simulink library "ConverterLibrary"  (R2026a)
settings: Solver=VariableStepAuto
undefined symbols (not defined in the file or in its folder): DiscIntNeverNeededParam, dspblkCoreblockFVToolHelper, gcbh, gridInverter
libraries: fl_lib x240, nesl_utility x221, ee_lib x208, slpidlib x28, eeGeneralControl x12, simulink x9, eeTransforms x4, simulink_extras x1, eePowerMeasurement x1
(part 3 of 30)

== system ConverterLibrary/Power Converter Plant/Power Factor Correction Converters ==
  Boost PFC Converter : Subsystem  mask(Boost PFC Converter){modelOption=Simplified, ratedPower=1000, ratedPower_unit=W, VIn=230, VIn_unit=V, FRated=50, FRated_unit=Hz, VOut=400, VOut_unit=V, Fsw=65000, Fsw_unit=Hz, LBoost=9.5731e-4, LBoost_unit=H, RLboost=0.05, RLboost_unit=Ohm, CBoost=7.9577e-4, CBoost_unit=F, Rco=0.01, Rco_unit=Ohm, Vco=380, Vco_unit=V, switchDeviceOption=MOSFET (Ideal, Switching) with Thermal, RdsOn=0.05, RdsOn_unit=Ohm, GdsOff=1e-5, GdsOff_unit=1/Ohm, Vth=3, Vth_unit=V, diodeDeviceOption=Tabulated Diode, VfDiode=0.6, VfDiode_unit=V, RdDiode=0.01, RdDiode_unit=Ohm, GdDiode=1e-5, GdDiode_unit=1/Ohm, rectDiodeDeviceOption=Tabulated Diode, VfRect=0.6, VfRect_unit=V, RdRect=0.3, RdRect_unit=Ohm, GdRect=1e-5, GdRect_unit=1/Ohm, VfPreCharge=0.6, VfPreCharge_unit=V, RdPreCharge=0.01, RdPreCharge_unit=Ohm, GdPreCharge=1e-5, GdPreCharge_unit=1/Ohm, RPreCharge=3, RPreCharge_unit=Ohm, simTemp=25, simTemp_unit=degC}
      mask prompts: modelOption "Boost PFC model option"; ratedPower "Rated power"; VIn "AC input voltage (RMS)"; FRated "Line frequency"; VOut "DC output voltage"; Fsw "Switching frequency"; LBoost "Boost inductance"; RLboost "Inductor resistance"; CBoost "Output capacitance"; Rco "Capacitor ESR"; Vco "Initial output capacitor voltage"; switchDeviceOption "Switch model"; RdsOn "On-state resistance"; GdsOff "Off-state conductance"; Vth "Threshold voltage"; diodeDeviceOption "Diode model"; VfDiode "Forward voltage"; RdDiode "On resistance"; GdDiode "Off conductance"; rectDiodeDeviceOption "Rectifier diode model"; VfRect "Forward voltage"; RdRect "On resistance"; GdRect "Off conductance"; VfPreCharge "Forward voltage"; RdPreCharge "On resistance"; GdPreCharge "Off conductance"; RPreCharge "Pre-charge resistance"; simTemp "Simulation temperature"
      mask help: Single-phase diode bridge + boost PFC power stage
      mask init:
      | %% Unit conversion: convert displayed values to base SI units
      | convMap = containers.Map( ...
      |     {'W','kW','MW','V','kV','mV','F','mF','uF','nF','pF', ...
      |      'H','mH','uH','nH','Ohm','kOhm','mOhm','S','mS','1/Ohm', ...
      |      'Hz','kHz','MHz'}, ...
      |     {1, 1e3, 1e6, 1, 1e3, 1e-3, 1, 1e-3, 1e-6, 1e-9, 1e-12, ...
      |      1, 1e-3, 1e-6, 1e-9, 1, 1e3, 1e-3, 1, 1e-3, 1, ...
      |      1, 1e3, 1e6});
      | 
      | ratedPower_SI = ratedPower * convMap(ratedPower_unit);
      | VIn_SI = VIn * convMap(VIn_unit);
      | FRated_SI = FRated * convMap(FRated_unit);
      | VOut_SI = VOut * convMap(VOut_unit);
      | Fsw_SI = Fsw * convMap(Fsw_unit);
      | LBoost_SI = LBoost * convMap(LBoost_unit);
      | RLboost_SI = RLboost * convMap(RLboost_unit);
      | CBoost_SI = CBoost * convMap(CBoost_unit);
      | Rco_SI = Rco * convMap(Rco_unit);
      | Vco_SI = Vco * convMap(Vco_unit);
      | RdsOn_SI = RdsOn * convMap(RdsOn_unit);
      | GdsOff_SI = GdsOff * convMap(GdsOff_unit);
      | Vth_SI = Vth * convMap(Vth_unit);
      | VfDiode_SI = VfDiode * convMap(VfDiode_unit);
      | RdDiode_SI = RdDiode * convMap(RdDiode_unit);
      | GdDiode_SI = GdDiode * convMap(GdDiode_unit);
      | 
      | 
      | VfRect_SI = VfRect * convMap(VfRect_unit);
      | RdRect_SI = RdRect * convMap(RdRect_unit);
      | GdRect_SI = GdRect * convMap(GdRect_unit);
      | % Pre-charge circuit parameters
      | VfPreCharge_SI = VfPreCharge * convMap(VfPreCharge_unit);
      | RdPreCharge_SI = RdPreCharge * convMap(RdPreCharge_unit);
      | GdPreCharge_SI = GdPreCharge * convMap(GdPreCharge_unit);
      | RPreCharge_SI = RPreCharge * convMap(RPreCharge_unit);
      | 
      | 
      | %% Simulation temperature (thermal MOSFET and tabulated diodes)
      | % Temperature is an OFFSET unit (K = degC + 273.15), so it cannot use the
      | % multiplicative convMap above; convert it explicitly. simTemp_K is read directly by
      | % the thermal MOSFET junction-temperature target, by the boost switch's Temperature Source, and by
      | % every tabulated diode's device simulation temperature.
      | if strcmp(simTemp_unit, 'degC')
      |     simTemp_K = simTemp + 273.15;
      | else
      |     simTemp_K = simTemp;
      | end
      | 
      | %% Apply variant selection
      | selectBoostPFCModelOption(gcb);
      settings: CopyFcn="set_param(gcbh,\"LinkStatus\",\"none\");"  PortSchema="{\"entries\":[{\"content\":{\"sides\":[{\"content\":{\"connectorIds\":[\"LConn1\",\"LConn2\"]},\"type\":\"ConnectorPlacement.EquallySpacedRectSide\",\"uuid\":\"1dbc8d27-ad96-467a-a357-3fb6b54f5038\"},{\"content\":{\"connectorIds\":[\"RConn1\",\"RConn2\"],\"side\":\"RIGHT\"},\"type\":\"ConnectorPlacement.EquallySpacedRectSide\",\"uuid\":\"a7801564-f46e-4876-bbd0-388b36974b7d\"},{\"content\":{\"connectorIds\":[\"In1\",\"Out1\"],\"side\":\"TOP\"},\"type\":\"ConnectorPlacement.EquallySpacedRectSide\",\"uuid\":\"b9e6132f-a5e8-4db3-b298-fdce73dc02b1\"}]},\"type\":\"ConnectorPlacement.EquallySpacedConnector\",\"uuid\":\"f45ea93c-581d-4ac6-a344-7b31d290ff6c\"}],\"packageUris\":[\"http://schema.mathworks.com/mf0/Connector/R2020b\"],\"version\":\"1.0\"}"
      mask Help: web('BoostPFC.html')
      mask TypeOptions modelOption: Simplified | Detailed
      mask Callback modelOption: selectBoostPFCModelOption(gcb);
      mask TypeOptions ratedPower_unit: W | kW | MW
      mask TypeOptions VIn_unit: V | kV | mV
      mask TypeOptions FRated_unit: Hz | kHz
      mask TypeOptions VOut_unit: V | kV | mV
      mask TypeOptions Fsw_unit: Hz | kHz | MHz
      mask TypeOptions LBoost_unit: H | mH | uH
      mask TypeOptions RLboost_unit: Ohm | kOhm | mOhm
      mask TypeOptions CBoost_unit: F | mF | uF | nF
      mask TypeOptions Rco_unit: Ohm | kOhm | mOhm
      mask TypeOptions Vco_unit: V | kV | mV
      mask TypeOptions switchDeviceOption: Ideal Switch | MOSFET (Ideal, Switching) with Thermal
      mask Callback switchDeviceOption: selectBoostPFCSwitchDevice(gcb);
      mask TypeOptions RdsOn_unit: Ohm | kOhm | mOhm
      mask TypeOptions GdsOff_unit: 1/Ohm | S | mS
      mask TypeOptions Vth_unit: V | kV | mV
      mask TypeOptions diodeDeviceOption: Ideal Diode | Tabulated Diode
      mask Callback diodeDeviceOption: selectBoostPFCDiodeDevice(gcb);
      mask TypeOptions VfDiode_unit: V | kV | mV
      mask TypeOptions RdDiode_unit: Ohm | kOhm | mOhm
      mask TypeOptions GdDiode_unit: 1/Ohm | S | mS
      mask TypeOptions rectDiodeDeviceOption: Ideal Diode | Tabulated Diode
      mask Callback rectDiodeDeviceOption: selectBoostPFCRectifierDiodeDevice(gcb);
      mask TypeOptions VfRect_unit: V | mV | kV
      mask TypeOptions RdRect_unit: Ohm | mOhm | kOhm
      mask TypeOptions GdRect_unit: 1/Ohm
      mask TypeOptions VfPreCharge_unit: V | kV | mV
      mask TypeOptions RdPreCharge_unit: Ohm | kOhm | mOhm
      mask TypeOptions GdPreCharge_unit: 1/Ohm | S | mS
      mask TypeOptions RPreCharge_unit: Ohm | kOhm | mOhm
      mask TypeOptions simTemp_unit: degC | K
      mask DialogControl BoostPFCConverterParameters Prompt: Boost PFC Converter Parameters
      mask DialogControl SwitchDevice Prompt: Boost Stage Devices
      mask DialogControl openMOSFETMask Prompt: Open MOSFET block mask
      mask DialogControl openMOSFETMask Callback: open_system([gcb '/BoostPFCVariant/DetailedModel/BoostSwitch/SwitchingMOSFETwithThermal/MOSFET'], 'mask');
      mask DialogControl DiodeDevice Prompt: Boost Diode Device
      mask DialogControl openDiodeMask Prompt: Open Diode block mask
      mask DialogControl openDiodeMask Callback: open_system([gcb '/BoostPFCVariant/DetailedModel/BoostDiode/TabulatedDiode/Diode1'], 'mask');
      mask DialogControl RectifierDevices Prompt: Rectifier Devices
      mask DialogControl openRectDiodeMask Prompt: Open Rectifier Diode Mask
      mask DialogControl openRectDiodeMask Callback: open_system([gcb '/BoostPFCVariant/DetailedModel/RectifierBridge/TabulatedDiode/Diode1'], 'mask');
      mask DialogControl applyRectDiodeParam Prompt: Apply to All Rectifier Diodes
      mask DialogControl applyRectDiodeParam Callback: applyBoostPFCRectifierDiodeParameters(gcb);
      mask DialogControl PreChargeCircuit Prompt: Pre-Charge Circuit Parameters
      mask DialogControl ExportPanel Prompt: Export to Unmasked Subsystem
      mask DialogControl ExportInfo Prompt: To customize the converter, export it as an unmasked subsystem with the active variant flattened - a standalone, fully-editable circuit plus a parameter file. Requires the "Variant Manager for Simulink" add-on.
      mask DialogControl exportToModel Prompt: Export
      mask DialogControl exportToModel Callback: exportConverterModelFromMask(gcb);
      mask Display: image('BoostPFCDiodeIcon.svg');
  Interleaved Boost PFC Converter : Subsystem  mask(Interleaved Boost PFC Converter){modelOption=Simplified, ratedPower=2000, ratedPower_unit=W, VIn=230, VIn_unit=V, FRated=50, FRated_unit=Hz, VOut=400, VOut_unit=V, Fsw=65000, Fsw_unit=Hz, LBoost=9.5731e-4, LBoost_unit=H, RLboost=0.03, RLboost_unit=Ohm, CBoost=7.9577e-4, CBoost_unit=F, Rco=0.01, Rco_unit=Ohm, Vco=360, Vco_unit=V, switchDeviceOption=MOSFET (Ideal, Switching) with Thermal, RdsOn=0.05, RdsOn_unit=Ohm, GdsOff=1e-5, GdsOff_unit=1/Ohm, Vth=3, Vth_unit=V, simTemp=25, simTemp_unit=degC, diodeDeviceOption=Tabulated Diode, VfDiode=0.6, VfDiode_unit=V, RdDiode=0.01, RdDiode_unit=Ohm, GdDiode=1e-5, GdDiode_unit=1/Ohm, rectDiodeDeviceOption=Tabulated Diode, VfRect=0.7, VfRect_unit=V, RdRect=0.01, RdRect_unit=Ohm, GdRect=1e-5, GdRect_unit=S, VfPreCharge=0.6, VfPreCharge_unit=V, RdPreCharge=0.01, RdPreCharge_unit=Ohm, GdPreCharge=1e-5, GdPreCharge_unit=1/Ohm, RPreCharge=3, RPreCharge_unit=Ohm}
      mask prompts: modelOption "Interleaved Boost PFC model option"; ratedPower "Rated power"; VIn "AC input voltage (RMS)"; FRated "Line frequency"; VOut "DC output voltage"; Fsw "Switching frequency"; LBoost "Phase inductance"; RLboost "Inductor resistance"; CBoost "Output capacitance"; Rco "Capacitor ESR"; Vco "Initial output capacitor voltage"; switchDeviceOption "Switch model"; RdsOn "On-state resistance"; GdsOff "Off-state conductance"; Vth "Threshold voltage"; simTemp "Simulation temperature"; diodeDeviceOption "Diode model"; VfDiode "Forward voltage"; RdDiode "On resistance"; GdDiode "Off conductance"; rectDiodeDeviceOption "Rectifier diode model"; VfRect "Forward voltage"; RdRect "On resistance"; GdRect "Off conductance"; VfPreCharge "Forward voltage"; RdPreCharge "On resistance"; GdPreCharge "Off conductance"; RPreCharge "Pre-charge resistance"
      mask help: Single-phase diode bridge + 2-phase interleaved boost PFC
      mask init:
      | %% Unit conversion: convert displayed values to base SI units
      | convMap = containers.Map( ...
      |     {'W','kW','MW','V','kV','mV','F','mF','uF','nF','pF', ...
      |      'H','mH','uH','nH','Ohm','kOhm','mOhm','S','mS','1/Ohm', ...
      |      'Hz','kHz','MHz'}, ...
      |     {1, 1e3, 1e6, 1, 1e3, 1e-3, 1, 1e-3, 1e-6, 1e-9, 1e-12, ...
      |      1, 1e-3, 1e-6, 1e-9, 1, 1e3, 1e-3, 1, 1e-3, 1, ...
      |      1, 1e3, 1e6});
      | 
      | ratedPower_SI = ratedPower * convMap(ratedPower_unit);
      | VIn_SI = VIn * convMap(VIn_unit);
      | FRated_SI = FRated * convMap(FRated_unit);
      | VOut_SI = VOut * convMap(VOut_unit);
      | Fsw_SI = Fsw * convMap(Fsw_unit);
      | LBoost_SI = LBoost * convMap(LBoost_unit);
      | RLboost_SI = RLboost * convMap(RLboost_unit);
      | CBoost_SI = CBoost * convMap(CBoost_unit);
      | Rco_SI = Rco * convMap(Rco_unit);
      | Vco_SI = Vco * convMap(Vco_unit);
      | RdsOn_SI = RdsOn * convMap(RdsOn_unit);
      | GdsOff_SI = GdsOff * convMap(GdsOff_unit);
      | Vth_SI = Vth * convMap(Vth_unit);
      | VfDiode_SI = VfDiode * convMap(VfDiode_unit);
      | RdDiode_SI = RdDiode * convMap(RdDiode_unit);
      | GdDiode_SI = GdDiode * convMap(GdDiode_unit);
      | VfRect_SI = VfRect * convMap(VfRect_unit);
      | RdRect_SI = RdRect * convMap(RdRect_unit);
      | GdRect_SI = GdRect * convMap(GdRect_unit);
      | % Pre-charge circuit parameters
      | VfPreCharge_SI = VfPreCharge * convMap(VfPreCharge_unit);
      | RdPreCharge_SI = RdPreCharge * convMap(RdPreCharge_unit);
      | GdPreCharge_SI = GdPreCharge * convMap(GdPreCharge_unit);
      | RPreCharge_SI = RPreCharge * convMap(RPreCharge_unit);
      | 
      | 
      | %% Simulation temperature (thermal MOSFET and tabulated diodes)
      | % Temperature is an OFFSET unit (K = degC + 273.15), so it cannot use the
      | % multiplicative convMap above; convert it explicitly. simTemp_K is read directly by
      | % the thermal MOSFET junction-temperature target, by each leg's Temperature Source, and by
      | % every tabulated diode's device simulation temperature.
      | if strcmp(simTemp_unit, 'degC')
      |     simTemp_K = simTemp + 273.15;
      | else
      |     simTemp_K = simTemp;
      | end
      | 
      | %% Apply variant selection
      | selectInterleavedBoostPFCModelOption(gcb);
      settings: CopyFcn="set_param(gcbh,\"LinkStatus\",\"none\");"  PortSchema="{\"entries\":[{\"content\":{\"sides\":[{\"content\":{\"connectorIds\":[\"LConn1\",\"LConn2\"]},\"type\":\"ConnectorPlacement.EquallySpacedRectSide\",\"uuid\":\"66face99-db51-4944-b334-77824ed81f08\"},{\"content\":{\"connectorIds\":[\"RConn1\",\"RConn2\"],\"side\":\"RIGHT\"},\"type\":\"ConnectorPlacement.EquallySpacedRectSide\",\"uuid\":\"9e52168e-0663-44af-82f2-191b03a2477e\"},{\"content\":{\"connectorIds\":[\"In1\",\"Out1\"],\"side\":\"TOP\"},\"type\":\"ConnectorPlacement.EquallySpacedRectSide\",\"uuid\":\"fee1f90d-1881-492b-99ff-2bc4ebcb726f\"}]},\"type\":\"ConnectorPlacement.EquallySpacedConnector\",\"uuid\":\"1b108626-23b3-4c50-a934-41566cfe725a\"}],\"packageUris\":[\"http://schema.mathworks.com/mf0/Connector/R2020b\"],\"version\":\"1.0\"}"
      mask Help: web('InterleavedBoostPFC.html')
      mask TypeOptions modelOption: Simplified | Detailed
      mask Callback modelOption: selectInterleavedBoostPFCModelOption(gcb);
      mask TypeOptions ratedPower_unit: W | kW | MW
      mask TypeOptions VIn_unit: V | kV | mV
      mask TypeOptions FRated_unit: Hz | kHz
      mask TypeOptions VOut_unit: V | kV | mV
      mask TypeOptions Fsw_unit: Hz | kHz | MHz
      mask TypeOptions LBoost_unit: H | mH | uH
      mask TypeOptions RLboost_unit: Ohm | kOhm | mOhm
      mask TypeOptions CBoost_unit: F | mF | uF | nF
      mask TypeOptions Rco_unit: Ohm | kOhm | mOhm
      mask TypeOptions Vco_unit: V | kV | mV
      mask TypeOptions switchDeviceOption: Ideal Switch | MOSFET (Ideal, Switching) with Thermal
      mask Callback switchDeviceOption: selectInterleavedBoostPFCSwitchDevice(gcb);
      mask TypeOptions RdsOn_unit: Ohm | kOhm | mOhm
      mask TypeOptions GdsOff_unit: 1/Ohm | S | mS
      mask TypeOptions Vth_unit: V | kV | mV
      mask TypeOptions simTemp_unit: degC | K
      mask TypeOptions diodeDeviceOption: Ideal Diode | Tabulated Diode
      mask Callback diodeDeviceOption: selectInterleavedBoostPFCDiodeDevice(gcb);
      mask TypeOptions VfDiode_unit: V | kV | mV
      mask TypeOptions RdDiode_unit: Ohm | kOhm | mOhm
      mask TypeOptions GdDiode_unit: 1/Ohm | S | mS
      mask TypeOptions rectDiodeDeviceOption: Ideal Diode | Tabulated Diode
      mask Callback rectDiodeDeviceOption: selectInterleavedBoostPFCRectifierDiodeDevice(gcb);
      mask TypeOptions VfRect_unit: V | mV
      mask TypeOptions RdRect_unit: Ohm | mOhm | kOhm
      mask TypeOptions GdRect_unit: S | mS | 1/Ohm
      mask TypeOptions VfPreCharge_unit: V | kV | mV
      mask TypeOptions RdPreCharge_unit: Ohm | kOhm | mOhm
      mask TypeOptions GdPreCharge_unit: 1/Ohm | S | mS
      mask TypeOptions RPreCharge_unit: Ohm | kOhm | mOhm
      mask DialogControl InterleavedBoostPFCConverterParameters Prompt: Interleaved Boost PFC Converter Parameters
      mask DialogControl SwitchDevice Prompt: Boost Stage Devices
      mask DialogControl openMOSFETMask Prompt: Open MOSFET block mask
      mask DialogControl openMOSFETMask Callback: open_system([gcb '/InterleavedBoostPFCVariant/DetailedModel/BoostSwitch1/SwitchingMOSFETwithThermal/MOSFET'], 'mask');
      mask DialogControl applyMOSFETParam Prompt: Apply parameters to all MOSFET blocks
      mask DialogControl applyMOSFETParam Callback: applyInterleavedMOSFETParameters(gcb)
      mask DialogControl DiodeDevice Prompt: Boost Diode Device
      mask DialogControl openDiodeMask Prompt: Open Diode block mask
      mask DialogControl openDiodeMask Callback: open_system([gcb '/InterleavedBoostPFCVariant/DetailedModel/BoostDiode1/TabulatedDiode/Diode1'], 'mask');
      mask DialogControl applyDiodeParam Prompt: Apply parameters to all Diode blocks
      mask DialogControl applyDiodeParam Callback: applyInterleavedDiodeParameters(gcb)
      mask DialogControl RectifierDevices Prompt: Rectifier Devices
      mask DialogControl openRectDiodeMask Prompt: Open Rectifier Diode Mask
      mask DialogControl openRectDiodeMask Callback: open_system([gcb '/InterleavedBoostPFCVariant/DetailedModel/RectifierBridge/TabulatedDiode/Diode1'], 'mask');
      mask DialogControl applyRectDiodeParam Prompt: Apply to All Rectifier Diodes
      mask DialogControl applyRectDiodeParam Callback: applyInterleavedRectifierDiodeParameters(gcb);
      mask DialogControl PreChargeCircuit Prompt: Pre-Charge Circuit Parameters
      mask DialogControl ExportPanel Prompt: Export to Unmasked Subsystem
      mask DialogControl ExportInfo Prompt: To customize the converter, export it as an unmasked subsystem with the active variant flattened - a standalone, fully-editable circuit plus a parameter file. Requires the "Variant Manager for Simulink" add-on.
      mask DialogControl exportToModel Prompt: Export
      mask DialogControl exportToModel Callback: exportConverterModelFromMask(gcb);
      mask Display: image('InterleavedBoostPFCDiodeIcon.svg');
  Totem-Pole Boost PFC Converter : Subsystem  mask(Totem-Pole Boost PFC Converter){modelOption=Simplified, ratedPower=3000, ratedPower_unit=W, VIn=230, VIn_unit=V, FRated=50, FRated_unit=Hz, VOut=400, VOut_unit=V, Fsw=100000, Fsw_unit=Hz, LBoost=2.0742e-4, LBoost_unit=H, RLboost=0.02, RLboost_unit=Ohm, CBoost=1.1937e-3, CBoost_unit=F, Rco=0.01, Rco_unit=Ohm, Vco=400, Vco_unit=V, fastLegDeviceOption=MOSFET (Ideal, Switching) with Thermal, RdsOnFast=0.04, RdsOnFast_unit=Ohm, GdsOffFast=1e-5, GdsOffFast_unit=1/Ohm, VthFast=3, VthFast_unit=V, simTempFast=25, simTempFast_unit=degC, slowLegDeviceOption=MOSFET, slowMOSFETDeviceOption=MOSFET (Ideal, Switching) with Thermal, slowDiodeDeviceOption=Ideal Diode, RdsOnSlow=0.05, RdsOnSlow_unit=Ohm, GdsOffSlow=1e-5, GdsOffSlow_unit=1/Ohm, VthSlow=3, VthSlow_unit=V, simTempSlow=25, simTempSlow_unit=degC, VfSlow=0.6, VfSlow_unit=V, RdSlow=0.01, RdSlow_unit=Ohm, GdSlow=1e-05, GdSlow_unit=1/Ohm, IhSlow=1, IhSlow_unit=A, VfFast=0.8, VfFast_unit=V, RdFast=0.001, RdFast_unit=Ohm, GdFast=1e-5, GdFast_unit=1/Ohm}
      mask prompts: modelOption "Totem-Pole Boost PFC Model Option"; ratedPower "Rated Power"; VIn "AC Input Voltage (RMS)"; FRated "Line Frequency"; VOut "DC Output Voltage"; Fsw "Switching Frequency"; LBoost "Boost Inductance"; RLboost "Inductor resistance"; CBoost "Output Capacitance"; Rco "Capacitor ESR"; Vco "Initial Output Capacitor Voltage"; fastLegDeviceOption "Fast Leg Device"; RdsOnFast "On-State Resistance"; GdsOffFast "Off-State Conductance"; VthFast "Threshold Voltage"; simTempFast "Simulation temperature"; slowLegDeviceOption "Slow Leg Device"; slowMOSFETDeviceOption "MOSFET Device"; slowDiodeDeviceOption "Diode Device"; RdsOnSlow "On-State Resistance (MOSFET)"; GdsOffSlow "Off-State Conductance"; VthSlow "Threshold Voltage"; simTempSlow "Simulation temperature"; VfSlow "Forward Voltage (Diode)"; RdSlow "On Resistance (Diode)"; GdSlow "Off Conductance (Diode)"; IhSlow "Holding current (Ih)"; VfFast "Forward Voltage (Body Diode)"; RdFast "On Resistance (Body Diode)"; GdFast "Off Conductance (Body Diode)"
      mask help: Bridgeless totem-pole boost PFC with fast and slow legs
      mask init:
      | %% Unit conversion: convert displayed values to base SI units
      | convMap = containers.Map( ...
      |     {'W','kW','MW','V','kV','mV','A','mA','F','mF','uF','nF','pF', ...
      |      'H','mH','uH','nH','Ohm','kOhm','mOhm','S','mS','1/Ohm', ...
      |      'Hz','kHz','MHz'}, ...
      |     {1, 1e3, 1e6, 1, 1e3, 1e-3, 1, 1e-3, 1, 1e-3, 1e-6, 1e-9, 1e-12, ...
      |      1, 1e-3, 1e-6, 1e-9, 1, 1e3, 1e-3, 1, 1e-3, 1, ...
      |      1, 1e3, 1e6});
      | 
      | ratedPower_SI = ratedPower * convMap(ratedPower_unit);
      | VIn_SI = VIn * convMap(VIn_unit);
      | FRated_SI = FRated * convMap(FRated_unit);
      | VOut_SI = VOut * convMap(VOut_unit);
      | Fsw_SI = Fsw * convMap(Fsw_unit);
      | LBoost_SI = LBoost * convMap(LBoost_unit);
      | RLboost_SI = RLboost * convMap(RLboost_unit);
      | CBoost_SI = CBoost * convMap(CBoost_unit);
      | Rco_SI = Rco * convMap(Rco_unit);
      | Vco_SI = Vco * convMap(Vco_unit);
      | RdsOnFast_SI = RdsOnFast * convMap(RdsOnFast_unit);
      | GdsOffFast_SI = GdsOffFast * convMap(GdsOffFast_unit);
      | VthFast_SI = VthFast * convMap(VthFast_unit);
      | VfFast_SI = VfFast * convMap(VfFast_unit);
      | RdFast_SI = RdFast * convMap(RdFast_unit);
      | GdFast_SI = GdFast * convMap(GdFast_unit);
      | RdsOnSlow_SI = RdsOnSlow * convMap(RdsOnSlow_unit);
      | GdsOffSlow_SI = GdsOffSlow * convMap(GdsOffSlow_unit);
      | VthSlow_SI = VthSlow * convMap(VthSlow_unit);
      | VfSlow_SI = VfSlow * convMap(VfSlow_unit);
      | RdSlow_SI = RdSlow * convMap(RdSlow_unit);
      | GdSlow_SI = GdSlow * convMap(GdSlow_unit);
      | IhSlow_SI = IhSlow * convMap(IhSlow_unit);
      | 
      | %% Simulation temperature (thermal MOSFET and tabulated diode)
      | % Temperature is an OFFSET unit (K = degC + 273.15), so it cannot use the
      | % multiplicative convMap; convert it explicitly. These Kelvin variables are
      | % read directly by each thermal MOSFET junction-temperature target, by each leg's
      | % Temperature Source, and by the slow-leg tabulated diodes' device simulation
      | % temperature - the only temperature input those diodes have, since they carry no
      | % thermal port.
      | if strcmp(simTempFast_unit, 'degC')
      |     simTempFast_K = simTempFast + 273.15;
      | else
      |     simTempFast_K = simTempFast;
      | end
      | if strcmp(simTempSlow_unit, 'degC')
      |     simTempSlow_K = simTempSlow + 273.15;
      | else
      |     simTempSlow_K = simTempSlow;
      | end
      | 
      | %% Apply variant selection
      | selectTotemPolePFCModelOption(gcb);
      settings: CopyFcn="set_param(gcbh,\"LinkStatus\",\"none\");"  PortSchema="{\"entries\":[{\"content\":{\"sides\":[{\"content\":{\"connectorIds\":[\"LConn1\",\"LConn2\"]},\"type\":\"ConnectorPlacement.EquallySpacedRectSide\",\"uuid\":\"1524dc94-6d10-41c3-9c4d-140b0cbad198\"},{\"content\":{\"connectorIds\":[\"RConn1\",\"RConn2\"],\"side\":\"RIGHT\"},\"type\":\"ConnectorPlacement.EquallySpacedRectSide\",\"uuid\":\"3d33c594-269c-419c-bd3b-3274925b3c44\"},{\"content\":{\"connectorIds\":[\"In1\",\"Out1\"],\"side\":\"TOP\"},\"type\":\"ConnectorPlacement.EquallySpacedRectSide\",\"uuid\":\"36540d5a-957f-45fd-8e0e-0b298bd16df8\"}]},\"type\":\"ConnectorPlacement.EquallySpacedConnector\",\"uuid\":\"4eeec72c-6b37-4cf7-b4fd-97832ebea029\"}],\"packageUris\":[\"http://schema.mathworks.com/mf0/Connector/R2020b\"],\"version\":\"1.0\"}"
      mask Help: web('TotemPoleBoostPFC.html')
      mask TypeOptions modelOption: Simplified | Detailed
      mask Callback modelOption: selectTotemPolePFCModelOption(gcb);
      mask TypeOptions ratedPower_unit: W | kW | MW
      mask TypeOptions VIn_unit: V | kV | mV
      mask TypeOptions FRated_unit: Hz | kHz
      mask TypeOptions VOut_unit: V | kV | mV
      mask TypeOptions Fsw_unit: Hz | kHz | MHz
      mask TypeOptions LBoost_unit: H | mH | uH
      mask TypeOptions RLboost_unit: Ohm | kOhm | mOhm
      mask TypeOptions CBoost_unit: F | mF | uF | nF
      mask TypeOptions Rco_unit: Ohm | kOhm | mOhm
      mask TypeOptions Vco_unit: V | kV | mV
      mask TypeOptions fastLegDeviceOption: Ideal Switch | MOSFET (Ideal, Switching) with Thermal
      mask Callback fastLegDeviceOption: selectTotemPolePFCFastLeg(gcb);
      mask TypeOptions RdsOnFast_unit: Ohm | kOhm | mOhm
      mask TypeOptions GdsOffFast_unit: 1/Ohm | S | mS
      mask TypeOptions VthFast_unit: V | kV | mV
      mask TypeOptions simTempFast_unit: degC | K
      mask TypeOptions slowLegDeviceOption: Diode | MOSFET | Thyristor
      mask Callback slowLegDeviceOption: selectTotemPolePFCSlowLeg(gcb);
      mask TypeOptions slowMOSFETDeviceOption: Ideal Switch | MOSFET (Ideal, Switching) with Thermal
      mask Callback slowMOSFETDeviceOption: selectTotemPoleSlowMOSFETDevice(gcb);
      mask TypeOptions slowDiodeDeviceOption: Ideal Diode | Tabulated Diode
      mask Callback slowDiodeDeviceOption: selectTotemPoleSlowDiodeDevice(gcb);
      mask TypeOptions RdsOnSlow_unit: Ohm | kOhm | mOhm
      mask TypeOptions GdsOffSlow_unit: 1/Ohm | S | mS
      mask TypeOptions VthSlow_unit: V | kV | mV
      mask TypeOptions simTempSlow_unit: degC | K
      mask TypeOptions VfSlow_unit: V | kV | mV
      mask TypeOptions RdSlow_unit: Ohm | kOhm | mOhm
      mask TypeOptions GdSlow_unit: 1/Ohm | S | mS
      mask TypeOptions IhSlow_unit: A
      mask TypeOptions VfFast_unit: V | kV | mV
      mask TypeOptions RdFast_unit: Ohm | kOhm | mOhm
      mask TypeOptions GdFast_unit: 1/Ohm | S | mS
      mask DialogControl Totem_PoleBoostPFCConverterParameters Prompt: Totem-Pole Boost PFC Converter Parameters
      mask DialogControl FastLegDevice Prompt: Fast Leg Device
      mask DialogControl openFastMOSFETMask Prompt: Open MOSFET block mask
      mask DialogControl openFastMOSFETMask Callback: openTotemPoleDeviceMask(gcb, 'fastThermalMOSFET');
      mask DialogControl applyFastMOSFETParam Prompt: Apply parameters to all fast leg MOSFET blocks
      mask DialogControl applyFastMOSFETParam Callback: applyTotemPoleFastMOSFETParameters(gcb);
      mask DialogControl SlowLegDevice Prompt: Slow Leg Device
      mask DialogControl openSlowMOSFETMask Prompt: Open MOSFET block mask
      mask DialogControl openSlowMOSFETMask Callback: openTotemPoleDeviceMask(gcb, 'slowThermalMOSFET');
      mask DialogControl applySlowMOSFETParam Prompt: Apply parameters to all slow leg MOSFET blocks
      mask DialogControl applySlowMOSFETParam Callback: applyTotemPoleSlowMOSFETParameters(gcb);
      mask DialogControl openSlowDiodeMask Prompt: Open Diode block mask
      mask DialogControl openSlowDiodeMask Callback: openTotemPoleDeviceMask(gcb, 'slowTabulatedDiode');
      mask DialogControl applySlowDiodeParam Prompt: Apply parameters to all slow leg Diode blocks
      mask DialogControl applySlowDiodeParam Callback: applyTotemPoleSlowDiodeParameters(gcb);
      mask DialogControl ExportPanel Prompt: Export to Unmasked Subsystem
      mask DialogControl ExportInfo Prompt: To customize the converter, export it as an unmasked subsystem with the active variant flattened - a standalone, fully-editable circuit plus a parameter file. Requires the "Variant Manager for Simulink" add-on.
      mask DialogControl exportToModel Prompt: Export
      mask DialogControl exportToModel Callback: exportConverterModelFromMask(gcb);
      mask Display:
      | slowLeg = get_param(gcb, 'slowLegDeviceOption');
      | if strcmp(slowLeg, 'Diode')
      |     image('TotemPoleDiodeIcon.svg');
      | elseif strcmp(slowLeg, 'Thyristor')
      |     image('TotemPoleThyristorIcon.svg');
      | else
      |     image('TotemPoleMOSFETIcon.svg');
      | end
